simulink model "LAB3_CrazyFlie_2026_ros2_easy_new"  (R2024b)
settings: Solver=ode45  StartTime=0.0  StopTime=inf  MaxStep=0.1  RelTol=1e-3  EnableMultiTasking=on
PreLoadFcn:
  | % load parameters of the default quadrotor
  | disp('Quadrotor parameters loaded by PreLoadFcn')
  | mdl_quadrotor
undefined symbols (not defined in the file): angular, linear, rot2
libraries: ros2lib x3, simulink_extras x3
settings Model: Creator=corkep  LastModifiedBy=macie
settings SolverCC: AlgebraicLoopSolver=TrustRegion
settings DataIOCC: LimitDataPoints=on  ReturnWorkspaceOutputs=off
settings OptimizationCC: ReuseModelBlockBuffer=off  ExpressionDepthLimit=2147483647  LifeSpan=inf
settings DebuggingCC: UnderspecifiedInitializationDetection=Classic  MergeDetectMultiDrivingBlocksExec=none  SolverPrmCheckMsg=warning  UnconnectedInputMsg=warning  UnconnectedOutputMsg=warning  UnconnectedLineMsg=warning  AllowSymbolicDim=off  StateNameClashWarn=warning  SFUnexpectedBacktrackingDiag=warning  SFNoUnconditionalDefaultTransitionDiag=warning  SFExecutionAtInitializationDiag=none  ArithmeticOperatorsInVariantConditions=warning
settings HardwareCC: ProdBitPerPointer=32  ProdBitPerSizeT=32  ProdBitPerPtrDiffT=32  ProdLargestAtomicFloat=None  ProdIntDivRoundTo=Undefined  ProdEndianess=Unspecified  ProdWordSize=32  ProdHWDeviceType=32-bit Generic
settings ModelReferenceCC: EnableRefExpFcnMdlSchedulingChecks=on  PropagateSignalLabelsOutOfModel=off
settings SFSimCC: SimUseLocalCustomCode=off  CustomCodeUndefinedFunction=UseInterfaceOnly
settings RTWCC: RTWUseLocalCustomCode=off  GPUComputeCapability=3.5  DLArmComputeVersion=19.05
settings CodeAppCC: StateflowObjectComments=on
settings GRTTargetCC: TargetLangStandard=C89/C90 (ANSI)  CombineOutputUpdateFcns=off  GRTInterface=on
settings ConfigComp: CovMetricSettings=de  CovSaveCumulativeToWorkspaceVar=on  CovSaveSingleToWorkspaceVar=on  CovExternalEMLEnable=off  CovSFcnEnable=off  CovBoundaryAbsTol=1.0e-5

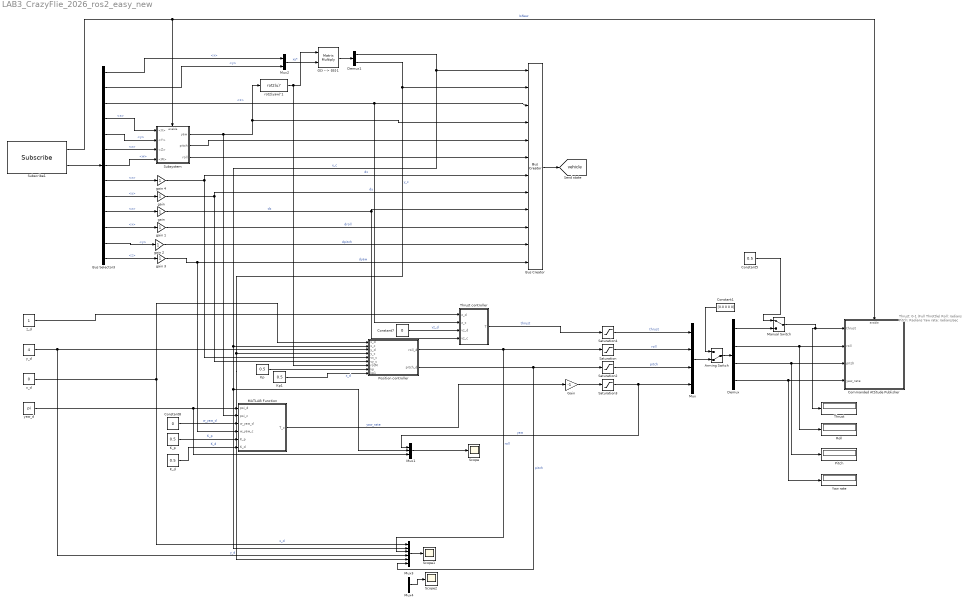
== system LAB3_CrazyFlie_2026_ros2_easy_new ==
  note: Thrust: 0-1 (Full Throttle)
      | Roll: radians
      | Pitch: Radians
      | Yaw rate: radians/sec
  Arming Switch : ManualSwitch  CurrentSetting=0
  Bus Creator : BusCreator  Inputs=12
  Bus Selector3 : BusSelector  OutputSignals=pose.pose.position.x,pose.pose.position.y,pose.pose.position.z,pose.pose.orientation.x,pose.pose.orientation.y,pose.pose.orientation.z,pose.pose.orientation.w,twist.twist.linear.x,twist.twist.linear.y,twist.twist.linear.z,twist.twist.angular.x,twist.twist.angular.y,twist.twist.angular.z
  Commanded Attitude Publisher : Subsystem
  Constant1 : Constant  Value=[0.0 0 0 0]
  Constant5 : Constant  Value=0.5
  Constant7 : Constant  Value=0
  Constant8 : Constant  Value=0
  Demux : Demux
  Demux1 : Demux  Outputs=2
  Gain : Gain  Gain=-1
  K_d : Constant  Value=0.5
  K_p : Constant  Value=0.5
  Kp : Constant  Value=0.5
  Kp1 : Constant  Value=0.5
  MATLAB Function : MATLAB Function  TreatAsAtomicUnit=on
  Manual Switch : ManualSwitch
  Mux : Mux
  Mux1 : Mux  Inputs=3
  Mux2 : Mux  Inputs=2
  Mux3 : Mux  Inputs=6
  Mux4 : Mux  Inputs=3
  Pitch : Display
  Position controller : MATLAB Function  TreatAsAtomicUnit=on
  Roll : Display
  Saturation : Saturate  UpperLimit=1  LowerLimit=-1
  Saturation2 : Saturate  UpperLimit=1  LowerLimit=-1
  Saturation3 : Saturate  UpperLimit=1  LowerLimit=-1
  Saturation4 : Saturate  UpperLimit=1  LowerLimit=0
  Scope : Scope
  Scope1 : Scope
  Scope2 : Scope
  Subscribe1 : ros2lib/Subscribe  topicSource=Select from ROS network  topic=/vicon/DEMO4/DEMO4/odom  messageType=nav_msgs/Odometry  SubscriberMode=At sample time  sampleTime=-1  CallbackGroupType=Default  CallbackGroupName=callback_group_1  QOSHistory=Keep last  QOSDepth=1  QOSReliability=Reliable  QOSDurability=Volatile  QOSDeadline=Inf  QOSLifespan=Inf  QOSLiveliness=Automatic  QOSLeaseDuration=Inf  QOSAvoidROSNamespaceConventions=off
  Subsystem : Subsystem
  Thrust : Display
  Thrust controller : MATLAB Function  TreatAsAtomicUnit=on
  Yaw rate : Display
  gain : Gain
  gain {,1..4} (5 alike) : Gain
  rot2(yaw)'1 : MATLABFcn  MATLABFcn=rot2(u)'  OutputDimensions=[2 2]  Output1D=off
  x_d : Constant  Value=0
  y_d : Constant  Value=4
  yaw_d : Constant  Value=pi
  z_d : Constant
  "{0} --> {B}1" : Product  Multiplication=Matrix(*)  RndMeth=Zero
  tag scope: vehicle=global
  wires:
  Bus Selector3/11 -> gain 1/1  "<x>"
  Bus Selector3/13 -> gain 3/1  "<z>"
  Bus Selector3/10 -> "gain "/1  "<z>"
  Bus Selector3/9 -> gain/1  "<y>"
  Bus Selector3/8 -> gain 4/1  "<x>"
  Bus Selector3/3 -> Thrust controller/2(z_c), Bus Creator/3  "<z>"
  Bus Creator/1 -> [vehicle]
  Bus Selector3/12 -> gain 2/1  "<y>"
  Subscribe1/2 -> Bus Selector3/1
  Mux2/1 -> "{0} --> {B}1"/2  "xy*"
  "{0} --> {B}1"/1 -> Demux1/1
  Demux1/1 -> Mux1/2, Mux3/2, Position controller/2(x_c), Bus Creator/1  "x_c"
  Demux1/2 -> Mux3/5, Position controller/4(y_c), Bus Creator/2  "y_c"
  Bus Selector3/2 -> Mux2/2  "<y>"
  rot2(yaw)'1/1 -> Position controller/7(rotM), "{0} --> {B}1"/1
  "gain "/1 -> Thrust controller/4(vz_c), Bus Creator/9  "dz"
  gain 1/1 -> Bus Creator/10  "droll"
  gain 2/1 -> Bus Creator/11  "dpitch"
  gain 3/1 -> MATLAB Function/4(w_yaw_c), Bus Creator/12  "dyaw"
  Subsystem/1(yaw) -> rot2(yaw)'1/1, Bus Creator/4, MATLAB Function/2(psi_c)
  Bus Selector3/4 -> Subsystem/1(<X>)  "<x>"
  Bus Selector3/5 -> Subsystem/2(<Y>)  "<y>"
  Bus Selector3/6 -> Subsystem/3(<Z>)  "<z>"
  Bus Selector3/7 -> Subsystem/4(<W>)  "<w>"
  Subsystem/2(pitch) -> Bus Creator/5
  Subsystem/3(roll) -> Bus Creator/6
  Bus Selector3/1 -> Mux2/1  "<x>"
  gain 4/1 -> Position controller/5(vx_c), Bus Creator/7  "dx"
  gain/1 -> Position controller/6(vy_c), Bus Creator/8  "dy"
  Subscribe1/1 -> Commanded Attitude Publisher/Enable, Subsystem/Enable  "IsNew"
  Demux/2 -> Roll/1, Commanded Attitude Publisher/2(roll)
  Demux/3 -> Pitch/1, Commanded Attitude Publisher/3(pitch)
  Demux/4 -> Yaw rate/1, Commanded Attitude Publisher/4(yaw_rate)
  Constant1/1 -> Arming Switch/1
  Arming Switch/1 -> Demux/1
  Mux/1 -> Arming Switch/2
  Thrust controller/1(T) -> Saturation4/1  "thrust"
  Position controller/1(roll_d) -> Mux3/3, Saturation/1  "roll"
  Position controller/2(pitch_d) -> Mux3/6, Saturation2/1  "pitch"
  MATLAB Function/1(T_z) -> Gain/1  "yaw_rate"
  Kp/1 -> Position controller/8(kp)
  x_d/1 -> Mux3/1, Position controller/1(x_d)  "x_d"
  y_d/1 -> Position controller/3(y_d), Mux3/4  "y_d"
  z_d/1 -> Thrust controller/1(z_d)
  Saturation/1 -> Mux/2  "roll"
  Saturation2/1 -> Mux/3  "pitch"
  Saturation3/1 -> Mux/4, Mux1/1  "yaw"
  Saturation4/1 -> Mux/1  "thrust"
  Demux/1 -> Manual Switch/2
  Manual Switch/1 -> Commanded Attitude Publisher/1(thrust), Thrust/1
  Constant5/1 -> Manual Switch/1
  yaw_d/1 -> MATLAB Function/1(psi_d), Mux1/3
  Gain/1 -> Saturation3/1
  Mux1/1 -> Scope/1
  Mux3/1 -> Scope1/1
  Mux4/1 -> Scope2/1
  Constant7/1 -> Thrust controller/3(vz_d)  "vz_d"
  Constant8/1 -> MATLAB Function/3(w_yaw_d)  "w_yaw_d"
  K_p/1 -> MATLAB Function/5(K_p)  "K_p"
  K_d/1 -> MATLAB Function/6(K_d)  "K_d"
  Kp1/1 -> Position controller/9(kp1)  "x_d"

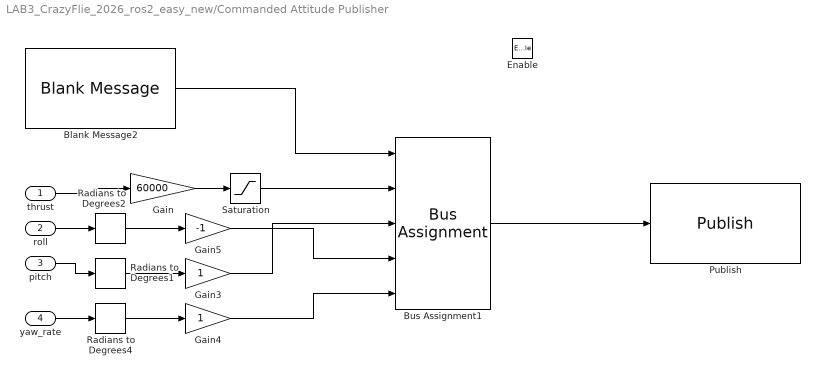
== system LAB3_CrazyFlie_2026_ros2_easy_new/Commanded Attitude Publisher ==
  thrust : Inport
  roll : Inport  Port=2
  pitch : Inport  Port=3
  yaw_rate : Inport  Port=4
  Enable : EnablePort
  Blank Message2 : ros2lib/Blank Message  messageClass=Message  entityType=geometry_msgs/Twist  messageType=geometry_msgs/Twist  SampleTime=1/30
  Bus Assignment1 : BusAssignment  DialogController=Simulink.DDGSource_BusAssignment  AssignedSignals=linear.z,linear.x,linear.y,angular.z
  Gain : Gain  Gain=60000
  Gain3 : Gain
  Gain4 : Gain
  Gain5 : Gain  Gain=-1
  Publish : ros2lib/Publish  topicSource=Select from ROS network  topic=/cf231/cmd_vel_legacy  messageType=geometry_msgs/Twist  QOSHistory=Keep last  QOSDepth=1  QOSReliability=Reliable  QOSDurability=Volatile  QOSDeadline=Inf  QOSLifespan=Inf  QOSLiveliness=Automatic  QOSLeaseDuration=Inf  QOSAvoidROSNamespaceConventions=off
  Radians to Degrees1 : simulink_extras/Transformations/Radians to Degrees
  Radians to Degrees2 : simulink_extras/Transformations/Radians to Degrees
  Radians to Degrees4 : simulink_extras/Transformations/Radians to Degrees
  Saturation : Saturate  UpperLimit=60000  LowerLimit=0
  wires:
  Bus Assignment1/1 -> Publish/1
  Blank Message2/1 -> Bus Assignment1/1
  thrust/1 -> Gain/1
  Gain/1 -> Saturation/1
  Saturation/1 -> Bus Assignment1/2
  Gain5/1 -> Bus Assignment1/4
  Radians to Degrees2/1 -> Gain5/1
  Radians to Degrees1/1 -> Gain3/1
  Radians to Degrees4/1 -> Gain4/1
  roll/1 -> Radians to Degrees2/1
  pitch/1 -> Radians to Degrees1/1
  Gain3/1 -> Bus Assignment1/3
  yaw_rate/1 -> Radians to Degrees4/1
  Gain4/1 -> Bus Assignment1/5

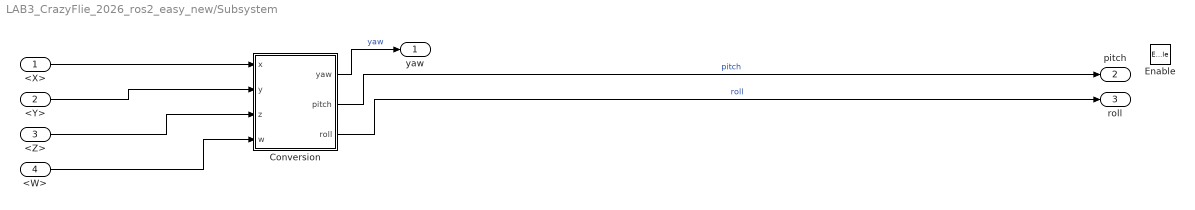
== system LAB3_CrazyFlie_2026_ros2_easy_new/Subsystem ==
  <X> : Inport
  <Y> : Inport  Port=2
  <Z> : Inport  Port=3
  <W> : Inport  Port=4
  Enable : EnablePort
  Conversion : MATLAB Function  TreatAsAtomicUnit=on
  yaw : Outport
  pitch : Outport  Port=2
  roll : Outport  Port=3
  wires:
  Conversion/1(yaw) -> yaw/1  "yaw"
  <X>/1 -> Conversion/1(x)
  Conversion/2(pitch) -> pitch/1  "pitch"
  <W>/1 -> Conversion/4(w)
  <Y>/1 -> Conversion/2(y)
  Conversion/3(roll) -> roll/1  "roll"
  <Z>/1 -> Conversion/3(z)

== matlab function LAB3_CrazyFlie_2026_ros2_easy_new/Subsystem/Conversion ==
  data: yaw output; x input; y input; z input; w input; pitch output; roll output
function [yaw,pitch,roll]  = quat2eul(x,y,z,w)
%#codegen

% Convert the quaternion to a yaw angle (zyx euler angle)
eul = quat2eul([w,x,y,z]);
yaw = eul(1);
roll = eul(3);
pitch = eul(2);

end

== matlab function LAB3_CrazyFlie_2026_ros2_easy_new/Position controller ==
  data: roll_d output; x_d input; x_c input; y_d input; pitch_d output; y_c input; vx_c input; vy_c input; rotM input; kp input; kp1 input
function [roll_d, pitch_d]  = fcn(x_d, x_c, y_d, y_c, vx_c, vy_c,rotM,kp,kp1)
   
    pos=[x_d,y_d]';
    pos=rotM*pos;
    x_d=pos(1);
    y_d=pos(2);
    ux_d = kp*(x_d - x_c);
    uy_d = kp*(y_d - y_c);

    pitch_d = kp1*(ux_d - vx_c);
    roll_d = kp1*(uy_d - vy_c);

== matlab function LAB3_CrazyFlie_2026_ros2_easy_new/Thrust controller ==
  data: z_d input; T output; z_c input; vz_d input; vz_c input
function T = fcn(z_d, z_c, vz_d, vz_c)
    kp = 0.1;
    kd = 0.1;
    T0 = 0.7;
    T = kp*(z_d - z_c) + kd*(vz_d-vz_c) + T0;

== matlab function LAB3_CrazyFlie_2026_ros2_easy_new/MATLAB Function ==
  data: psi_d input; T_z output; psi_c input; w_yaw_d input; w_yaw_c input; K_p input; K_d input
function T_z = fcn(psi_d,psi_c,w_yaw_d,w_yaw_c,K_p,K_d)



T_z=K_p*(wrapToPi(psi_d-psi_c))+K_d*(w_yaw_d-w_yaw_c);
